simulink model "Average_Model"  (R2025b)
settings: Solver=VariableStepAuto  StartTime=0.0  StopTime=inf  RelTol=1e-3
libraries: fl_lib x9, nesl_utility x7
settings Model: Creator=vivid  LastModifiedBy=vivid

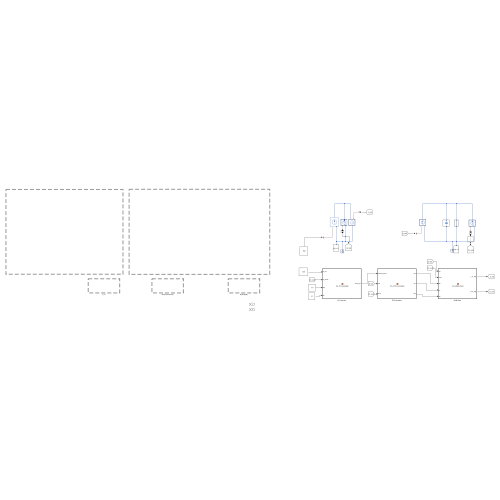
[thumbnail: Simulink's stored preview of the top-level diagram]
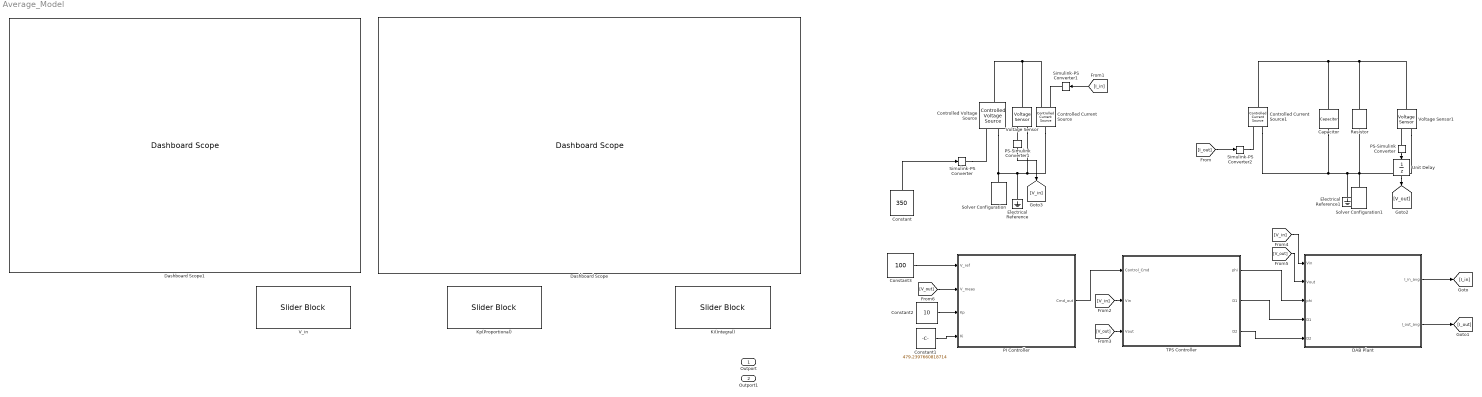
== system Average_Model ==
  Capacitor : fl_lib/Electrical/Electrical Elements/Capacitor  c=10 F  r=1e-6 Ohm  g=0 1/Ohm  i_specify=off  i_priority=None  i=0 A  i_nominal_specify=off  i_nominal_value=1  i_nominal_unit=A  v_specify=on  v_priority=None  v=10 V  v_nominal_specify=off  v_nominal_value=1  v_nominal_unit=V  vc_specify=off  vc_priority=High  vc=0 V  vc_nominal_specify=off  vc_nominal_value=1  vc_nominal_unit=V
  Constant : Constant  Value=350
  Constant1 : Constant  Value=479.2397660818714
  Constant2 : Constant  Value=10
  Constant3 : Constant  Value=100
  Controlled Current Source : fl_lib/Electrical/Electrical Sources/Controlled Current Source
  Controlled Current Source1 : fl_lib/Electrical/Electrical Sources/Controlled Current Source
  Controlled Voltage Source : fl_lib/Electrical/Electrical Sources/Controlled Voltage Source
  DAB Plant : MATLAB Function  TreatAsAtomicUnit=on
  Dashboard Scope : DashboardScope  FontColor=[0.0, 0.0, 0.0]
  Dashboard Scope1 : DashboardScope  Ymin=350  Ymax=450  FontColor=[0.0, 0.0, 0.0]
  Electrical Reference : fl_lib/Electrical/Electrical Elements/Electrical Reference
  Electrical Reference1 : fl_lib/Electrical/Electrical Elements/Electrical Reference
  Ki(Integral) : SliderBlock  ScaleMin=350  ScaleMax=1000
  Kp(Proportional) : SliderBlock  ScaleMax=10
  PI Controller : MATLAB Function  TreatAsAtomicUnit=on
  PS-Simulink Converter : nesl_utility/PS-Simulink Converter  PhysicalDomain=network_engine_domain  SubClassName=ps_output  LeftPortType=input  RightPortType=output  PseudoPeriodic=off  Frequencies=[]  VectorFormat=inherit  Unit=inherit  AffineConversion=off
  PS-Simulink Converter1 : nesl_utility/PS-Simulink Converter  PhysicalDomain=network_engine_domain  SubClassName=ps_output  LeftPortType=input  RightPortType=output  PseudoPeriodic=off  Frequencies=[]  VectorFormat=inherit  Unit=inherit  AffineConversion=off
  Resistor : fl_lib/Electrical/Electrical Elements/Resistor  R=100 Ohm  i_specify=off  i_priority=None  i=0 A  i_nominal_specify=off  i_nominal_value=1  i_nominal_unit=A  v_specify=on  v_priority=None  v=10 V  v_nominal_specify=off  v_nominal_value=1  v_nominal_unit=V
  Simulink-PS Converter : nesl_utility/Simulink-PS Converter  PhysicalDomain=network_engine_domain  SubClassName=ps_input  LeftPortType=input  RightPortType=output  PseudoPeriodic=off  Frequencies=[]  NoiseDistribution=none  NoiseParameters=[]  Unit=1  AffineConversion=off  FilteringAndDerivatives=provide  SimscapeFilterOrder=1  InputFilterTimeConstant=0.001  UdotUserProvided=0
  Simulink-PS Converter1 : nesl_utility/Simulink-PS Converter  PhysicalDomain=network_engine_domain  SubClassName=ps_input  LeftPortType=input  RightPortType=output  PseudoPeriodic=off  Frequencies=[]  NoiseDistribution=none  NoiseParameters=[]  Unit=1  AffineConversion=off  FilteringAndDerivatives=provide  SimscapeFilterOrder=1  InputFilterTimeConstant=0.001  UdotUserProvided=0
  Simulink-PS Converter2 : nesl_utility/Simulink-PS Converter  PhysicalDomain=network_engine_domain  SubClassName=ps_input  LeftPortType=input  RightPortType=output  PseudoPeriodic=off  Frequencies=[]  NoiseDistribution=none  NoiseParameters=[]  Unit=1  AffineConversion=off  FilteringAndDerivatives=provide  SimscapeFilterOrder=1  InputFilterTimeConstant=0.001  UdotUserProvided=0
  Solver Configuration : nesl_utility/Solver Configuration  PhysicalDomain=network_engine_domain  SubClassName=solver  LeftPortType=input  RightPortType=generic  Tones=[]  Harmonics=[]  SimulateNoise=off  Profile=off  UseLocalSampling=off  EnableSwitchedLinearOptims=on  FrequencyDomain=off  UseCCode=off  RelTol=0.001  AbsTol=0.001  MinStep=1e-09  ToWorkspace=off  RevertToSquareIcSolve=off  NumHomotopyIterations=100  PhasorMode=off  PhasorModeNumHarmonics=1  ConsistencySolver=NEWTON_XTOL_AFTER_FTOL  IndexReductionMethod=DerivativeReplacement  DoDC=off  ResidualTolerance=1e-09  ConsistencyTolSource=GLOBAL  ConsistencyAbsTol=0.001  ConsistencyRelTol=0.001  ConsistencyTolFactor=0.001  UseLocalSolver=off  LocalSolverChoice=NE_BACKWARD_EULER_ADVANCER  ResolveIndetEquations=on  FunctionEvalNumThread=1  LocalSolverSampleTime=0.001  DoFixedCost=off  MaxNonlinIter=3  MaxModeIter=2  ComputeImpulses=off  ImpulseIterations=2  LinearAlgebra=auto  LinearAlgebraNumThread=0  EquationFormulation=NE_TIME_EF  DelaysMemoryBudget=1024  AutomaticFiltering=on  FilteringTimeConstant=0.001  PartitionStorageMethod=AS_NEEDED  PartitionMemoryBudget=1024  PartitionMethod=ROBUST  MultibodyUseLocalSolver=off  MultibodyLocalSolverChoice=ODE1  MultibodyLocalSolverSampleTime=0.001
  Solver Configuration1 : nesl_utility/Solver Configuration  PhysicalDomain=network_engine_domain  SubClassName=solver  LeftPortType=input  RightPortType=generic  Tones=[]  Harmonics=[]  SimulateNoise=off  Profile=off  UseLocalSampling=off  EnableSwitchedLinearOptims=on  FrequencyDomain=off  UseCCode=off  RelTol=0.001  AbsTol=0.001  MinStep=1e-09  ToWorkspace=off  RevertToSquareIcSolve=off  NumHomotopyIterations=100  PhasorMode=off  PhasorModeNumHarmonics=1  ConsistencySolver=NEWTON_XTOL_AFTER_FTOL  IndexReductionMethod=DerivativeReplacement  DoDC=off  ResidualTolerance=1e-09  ConsistencyTolSource=GLOBAL  ConsistencyAbsTol=0.001  ConsistencyRelTol=0.001  ConsistencyTolFactor=0.001  UseLocalSolver=off  LocalSolverChoice=NE_BACKWARD_EULER_ADVANCER  ResolveIndetEquations=on  FunctionEvalNumThread=1  LocalSolverSampleTime=0.001  DoFixedCost=off  MaxNonlinIter=3  MaxModeIter=2  ComputeImpulses=off  ImpulseIterations=2  LinearAlgebra=auto  LinearAlgebraNumThread=0  EquationFormulation=NE_TIME_EF  DelaysMemoryBudget=1024  AutomaticFiltering=on  FilteringTimeConstant=0.001  PartitionStorageMethod=AS_NEEDED  PartitionMemoryBudget=1024  PartitionMethod=ROBUST  MultibodyUseLocalSolver=off  MultibodyLocalSolverChoice=ODE1  MultibodyLocalSolverSampleTime=0.001
  TPS Controller : MATLAB Function  TreatAsAtomicUnit=on
  Unit Delay : UnitDelay  SampleTime=-1  HasFrameUpgradeWarning=on
  V_in : SliderBlock  ScaleMin=350  ScaleMax=450
  Voltage Sensor : fl_lib/Electrical/Electrical Sensors/Voltage Sensor
  Voltage Sensor1 : fl_lib/Electrical/Electrical Sensors/Voltage Sensor
  Outport : Outport
  Outport1 : Outport  Port=2
  wires:
  PI Controller/1(Cmd_out) -> TPS Controller/1(Control_Cmd)
  TPS Controller/1(phi) -> DAB Plant/3(phi)
  TPS Controller/2(D1) -> DAB Plant/4(D1)
  TPS Controller/3(D2) -> DAB Plant/5(D2)
  DAB Plant/1(I_in_avg) -> [I_in]
  DAB Plant/2(I_out_avg) -> [I_out]
  [I_out] -> Simulink-PS Converter2/1
  [I_in] -> Simulink-PS Converter1/1
  PS-Simulink Converter1/1 -> [V_in]
  [V_in] -> TPS Controller/2(Vin)
  [V_out] -> TPS Controller/3(Vout)
  [V_out] -> DAB Plant/2(Vout)
  [V_in] -> DAB Plant/1(Vin)
  Unit Delay/1 -> [V_out]
  PS-Simulink Converter/1 -> Unit Delay/1
  [V_out] -> PI Controller/2(V_meas)
  Constant1/1 -> PI Controller/4(Ki)
  Constant2/1 -> PI Controller/3(Kp)
  Constant/1 -> Simulink-PS Converter/1
  Constant3/1 -> PI Controller/1(V_ref)
  connections:
  Simulink-PS Converter/RConn1 -- Controlled Voltage Source/RConn1
  Simulink-PS Converter2/RConn1 -- Controlled Current Source1/RConn1
  Simulink-PS Converter1/RConn1 -- Controlled Current Source/RConn1
  Controlled Voltage Source/RConn2 -- Solver Configuration/RConn1 -- Electrical Reference/LConn1 -- Controlled Current Source/LConn1 -- Voltage Sensor/RConn2
  Controlled Voltage Source/LConn1 -- Controlled Current Source/RConn2 -- Voltage Sensor/LConn1
  PS-Simulink Converter1/LConn1 -- Voltage Sensor/RConn1
  PS-Simulink Converter/LConn1 -- Voltage Sensor1/RConn1
  Capacitor/RConn1 -- Controlled Current Source1/RConn2 -- Resistor/RConn1 -- Voltage Sensor1/RConn2 -- Solver Configuration1/RConn1 -- Electrical Reference1/LConn1
  Controlled Current Source1/LConn1 -- Capacitor/LConn1 -- Resistor/LConn1 -- Voltage Sensor1/LConn1

== matlab function Average_Model/TPS Controller ==
  data: Control_Cmd input; phi output; Vin input; Vout input; D1 output; D2 output
function [phi, D1, D2] = fcn_TPS_Controller(Control_Cmd, Vin, Vout)
% TPS Optimization / Mapping Logic
% PI 제어기의 출력(Control_Cmd)을 받아 실제 스위칭 변수로 변환
% 향후 이 부분이 HDC(HyperDimensional Computing)나 LUT로 대체됩니다.

% 제한(Saturation) 설정
Cmd_Sat = min(max(Control_Cmd, -1), 1); % -1 ~ 1 사이로 제한

% --- 단순화된 TPS 전략 (예시) ---
% 전략: 부하가 적을 때는 D1, D2를 줄여 순환 전류(Reactive Power)를 줄이고,
% 부하가 클 때는 D1, D2를 최대로 하여 전력 전달을 극대화한다.

% 1. 위상각(phi) 계산: 주 전력 전달 제어 변수
% 최대 위상 0.5 (180도) 기준
phi = Cmd_Sat * 0.4; % 0.4(약 144도)까지만 사용 (안전 마진)

% 2. 듀티(D1, D2) 계산: 효율 최적화 변수
% 전력 지령(절대값)이 작으면 듀티를 줄임 (ZVS 보조 및 도통 손실 저감)
abs_cmd = abs(Cmd_Sat);

if abs_cmd > 0.6
    % 고부하 영역: PWM 폭 최대 (SPS 동작에 가까움)
    D1 = 0.5;
    D2 = 0.5;
elseif abs_cmd > 0.3
    % 중부하 영역: 듀티를 약간 줄임
    D1 = 0.4;
    D2 = 0.4;
else
    % 경부하 영역: 듀티를 많이 줄여 리플 전류 감소
    D1 = 0.25;
    D2 = 0.25;
end

% (선택) 전압비(k = V1/V2)에 따른 비대칭 듀티 제어
% if Vin > Vout ... end 식의 로직 추가 가능

end

== matlab function Average_Model/DAB Plant ==
  data: Vin input; I_in_avg output; Vout input; phi input; D1 input; D2 input; I_out_avg output
function [I_in_avg, I_out_avg] = fcn_DAB_Plant(Vin, Vout, phi, D1, D2)
% DAB Converter Average Model (Updated for Startup)

% -----------------------------------------------------------
% 1. 시스템 파라미터 설정
% -----------------------------------------------------------
L = 20e-6;      % 누설 인덕턴스 (20uH, 1차측 환산 기준)
fs = 100e3;     % 스위칭 주파수 (100kHz)
n = 4;          % [수정됨] 권선비 4:1 (입력 400V : 출력 100V 매칭)
loss_factor = 0.95; % 효율 95% 가정

% -----------------------------------------------------------
% 2. TPS 전력 전달 수식 계산
% -----------------------------------------------------------
% 분모 (임피던스 항)
denom = 2 * L * fs;

% 1차측으로 환산된 출력 전압 (Reflected Voltage)
% 물리적으로는 n * Vout이 1차측과 맞서 싸우는 전압입니다.
V_out_ref = n * Vout; 

if denom == 0
    P_transfer = 0;
else
    % 정규화된 위상차 절대값
    abs_phi = abs(phi);
    
    % SPS (Single Phase Shift) 기본 전력 수식
    % P = (V1 * V2) / (2*L*fs) * 4*phi*(0.5-|phi|)
    % 여기서 V2는 환산된 전압(V_out_ref)을 써야 합니다.
    k_sps = 4 * phi * (0.5 - abs_phi); 
    P_base = (Vin * V_out_ref) / denom * k_sps;
    
    % Duty Cycle Scaling (TPS 효과 근사화)
    % D1, D2가 0.5(최대)일 때 scaling = 1
    scaling = (D1 / 0.5) * (D2 / 0.5); 
    
    P_transfer = P_base * scaling;
end

% -----------------------------------------------------------
% 3. 입출력 평균 전류 계산 (핵심 수정 사항)
% -----------------------------------------------------------

% [입력 전류 계산]
if Vin > 1
    I_in_avg = P_transfer / Vin;
else
    I_in_avg = 0;
end

% [출력 전류 계산 - 초기 기동 문제 해결]
% 문제: Vout이 0이면 전류도 0이 되어 영원히 켜지지 않음 (Deadlock)
% 해결: 전압이 낮을 때는 강제로 '기동 전류'를 주입

if Vout < 5.0
    % [Soft Start] 전압이 5V 미만이면 수식 무시하고 5A 강제 주입
    % 커패시터를 충전시켜 0V를 탈출하게 함
    I_out_avg = 5.0; 
    
else
    % [정상 동작] P = V * I  =>  I = P / V
    % 0으로 나누기 방지를 위해 max(Vout, 1) 사용
    safe_Vout = max(Vout, 1.0);
    
    % 효율을 고려하여 출력 전류는 이론치보다 약간 적게 나감
    I_out_avg = (P_transfer * loss_factor) / safe_Vout;
end

end

== matlab function Average_Model/PI Controller ==
  data: V_ref input; Cmd_out output; V_meas input; Kp input; Ki input
function Cmd_out = fcn_PI_Controller(V_ref, V_meas, Kp, Ki)
% Discrete PI Controller with Anti-windup (Clamping)
% MCU 이식을 고려한 C-Style 코드입니다.

% --- 파라미터 설정 (튜닝 필요) ---
%Kp = 0.5;       % 비례 게인
%Ki = 500;       % 적분 게인
Ts = 50e-6;     % 제어 주기 (20kHz 가정)
Max_Out = 1.0;  % 출력 최대 제한
Min_Out = -1.0; % 출력 최소 제한

% --- 상태 변수 저장 (Persistent) ---
% C언어의 'static' 변수와 같습니다. 이전 값을 기억합니다.
persistent Integrator_Sum
if isempty(Integrator_Sum)
    Integrator_Sum = 0;
end

% 1. 오차 계산
Error = V_ref - V_meas;

% 2. 비례항 (P-term)
P_term = Kp * Error;

% 3. 적분항 (I-term) - 적분기 누적
% (임시로 더해보고 포화 여부 확인 예정)
Integrator_Sum_Next = Integrator_Sum + (Ki * Error * Ts);

% 4. 가출력 계산 (Pre-saturated Output)
Cmd_Pre = P_term + Integrator_Sum_Next;

% 5. Saturation 및 Anti-windup (Clamping 로직)
if Cmd_Pre > Max_Out
    Cmd_out = Max_Out;
    % 출력이 잘렸으므로, 적분기도 더 이상 쌓지 않음 (또는 제한된 값으로 유지)
    if Error > 0 
        % 에러가 여전히 양수면 적분기를 갱신하지 않음 (Clamping)
    else
        Integrator_Sum = Integrator_Sum_Next; % 에러가 줄어드는 방향이면 갱신 허용
    end
    
elseif Cmd_Pre < Min_Out
    Cmd_out = Min_Out;
    if Error < 0
        % Clamping
    else
        Integrator_Sum = Integrator_Sum_Next;
    end
    
else
    % 포화되지 않은 정상 구간
    Cmd_out = Cmd_Pre;
    Integrator_Sum = Integrator_Sum_Next; % 적분기 정상 누적
end

end
